simulink model "AlphaBotGyro"  (R2026b)
settings: Solver=FixedStepDiscrete  StopTime=inf  FixedStep=PAR_Sys_AbtastBasis_f64  EnableMultiTasking=on
StopFcn:
  | SpeichereGyroMessung('AlphaBotGyro');
model workspace (MAT data in the model file):
  PAR_AktMot_PWMLKreis_u8 = 60
  PAR_AktMot_PWMRKreis_u8 = 100
  PAR_AktMot_RichtL_u8 = 0
  PAR_AktMot_RichtR_u8 = 0
  PAR_AktMot_Start_f32 = Simulink.Parameter
  PAR_AktMot_Start_f32.Value = 0
  PAR_AktMot_Start_f32.Complexity = 'real'
  PAR_AktMot_Start_f32.Dimensions = [1 1]
  PAR_AktMot_Start_f32.DataType = 'single'
  PAR_RegKrs_TKreis_f64 = 10
  PAR_SenGyr_Abtast_f64 = 0.01
  PAR_SenGyr_NKalib_f64 = 1000
  PAR_Sys_AbtastBasis_f64 = 0.01
  PAR_Sys_Abtast_f64 = 0.01
libraries: arduinolib x6, arduinosensorlib x1
settings Model: SILPILModeSetting=veronly  SimulationMode=external
settings SolverCC: AutoInsertRateTranBlk=on
settings OptimizationCC: DifferentSizesBufferReuse=on  EfficientTunableParamExpr=on  EnhancedBackFolding=on  MaxStackSize=64  OptimizationCustomize=off  OptimizeBlockOrder=speed  PassReuseOutputArgsAs=Individual arguments  RemoveInternalMemoryZeroInit=on  RemoveRootLevelIOMemoryZeroInit=on
settings DebuggingCC: ParameterTunabilityLossMsg=error
settings HardwareCC: ProdHWDeviceType=ARM Compatible->ARM Cortex  ProdLargestAtomicFloat=Double  ProdLargestAtomicInteger=Long
settings SFSimCC: MATLABDynamicMemAlloc=off
settings RTWCC: BuildConfiguration=Faster Runs  Description=Embedded Coder  HardwareBoard=Arduino Uno R4 WiFi  SystemTargetFile=ert.tlc  TLCOptions=-aInlineSetEventsForThisBaseRateFcn=TLC_FALSE -aSuppressMultiTaskScheduler=TLC_FALSE -aRateBasedStepFcn=1  TemplateMakefile=ert_default_tmf  Toolchain=Arduino ARM M4
settings CodeAppCC: ForceParamTrailComments=on  IgnoreCustomStorageClasses=off  InsertBlockDesc=on  OperatorAnnotations=on  SFDataObjDesc=on  SimulinkDataObjDesc=on
settings ERTTargetCC: CombineSignalStateStructs=on  ExtModeAutomaticAllocSize=off  ExtModeIntrfLevel=Level2 - Open  ExtModeMexFile=ext_xcp  ExtModeStaticAlloc=on  SupportContinuousTime=on  SupportVariableSizeSignals=on

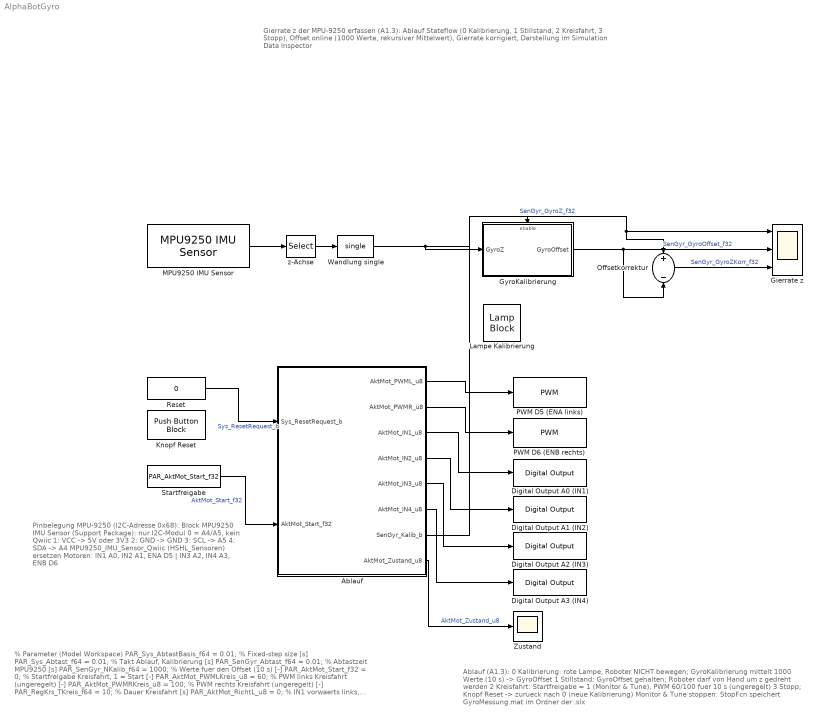
== system AlphaBotGyro ==
  note: % Parameter (Model Workspace)
      | PAR_Sys_AbtastBasis_f64 = 0.01; % Fixed-step size [s]
      | PAR_Sys_Abtast_f64 = 0.01; % Takt Ablauf, Kalibrierung [s]
      | PAR_SenGyr_Abtast_f64 = 0.01; % Abtastzeit MPU9250 [s]
      | PAR_SenGyr_NKalib_f64 = 1000; % Werte fuer den Offset (10 s) [-]
      | PAR_AktMot_Start_f32 = 0; % Startfreigabe Kreisfahrt, 1 = Start [-]
      | PAR_AktMot_PWMLKreis_u8 = 60; % PWM links Kreisfahrt (ungeregelt) [-]
      | PAR_AktMot_PWMRKreis_u8 = 100; % PWM rechts Kreisfahrt (ungeregelt) [-]
      | PAR_RegKrs_TKreis_f64 = 10; % Dauer Kreisfahrt [s]
      | PAR_AktMot_RichtL_u8 = 0; % IN1 vorwaerts links, IN2 = 1 - IN1 [-]
      | PAR_AktMot_RichtR_u8 = 1; % IN3 vorwaerts rechts, IN4 = 1 - IN3 [-]
  note: Gierrate z der MPU-9250 erfassen (A1.3): Ablauf Stateflow (0 Kalibrierung, 1 Stillstand, 2 Kreisfahrt, 3 Stopp), Offset online (1000 Werte, rekursiver Mittelwert), Gierrate korrigiert, Darstellung im Simulation Data Inspector
  note: Pinbelegung MPU-9250 (I2C-Adresse 0x68):
      | Block MPU9250 IMU Sensor (Support Package): nur I2C-Modul 0 = A4/A5, kein Qwiic
      | 1: VCC -> 5V oder 3V3
      | 2: GND -> GND
      | 3: SCL -> A5
      | 4: SDA -> A4
      | MPU9250_IMU_Sensor_Qwiic (HSHL_Sensoren) ersetzen
      | Motoren: IN1 A0, IN2 A1, ENA D5 | IN3 A2, IN4 A3, ENB D6
  note: Ablauf (A1.3):
      | 0 Kalibrierung: rote Lampe, Roboter NICHT bewegen; GyroKalibrierung mittelt 1000 Werte (10 s) -> GyroOffset
      | 1 Stillstand: GyroOffset gehalten; Roboter darf von Hand um z gedreht werden
      | 2 Kreisfahrt: Startfreigabe = 1 (Monitor & Tune), PWM 60/100 fuer 10 s (ungeregelt)
      | 3 Stopp; Knopf Reset -> zurueck nach 0 (neue Kalibrierung)
      | Monitor & Tune stoppen: StopFcn speichert GyroMessung.mat im Ordner der .slx
  Ablauf : Stateflow chart  TreatAsAtomicUnit=on
  Digital Output A0 (IN1) : arduinolib/Digital Output  pinNumber=14  Direction=output  blockPlatform=arduino
  Digital Output A1 (IN2) : arduinolib/Digital Output  pinNumber=15  Direction=output  blockPlatform=arduino
  Digital Output A2 (IN3) : arduinolib/Digital Output  pinNumber=16  Direction=output  blockPlatform=arduino
  Digital Output A3 (IN4) : arduinolib/Digital Output  pinNumber=17  Direction=output  blockPlatform=arduino
  Gierrate z : Scope  NumInputPorts=3
  GyroKalibrierung : Subsystem  TreatAsAtomicUnit=on
  Knopf Reset : PushButtonBlock  ButtonText=Reset  IconOnColor=[0.0, 0.39215686274509803, 0.0]  IconOffColor=[0.0, 1.0, 0.0]
  Lampe Kalibrierung : LampBlock  LabelPosition=Hide  DefaultColor=[192.0, 192.0, 192.0]
  MPU9250 IMU Sensor : arduinosensorlib/MPU9250 IMU Sensor  I2CModule=0  SlaveAddress=0x68  Accel=off  AngularRate=on  Ak8963Field=off  Temperature=off  Status=off  EulerAngles=off  Quat=off  Timestamp=off  AccelRange=2G  Acceldlpf=218.1 Hz  GyroRange=250 dps  Gyrodlpf=41 Hz  DmpOdr=200 Hz  spf=1  SampleTime=PAR_SenGyr_Abtast_f64  QueueSizeFactor=1
  Offsetkorrektur : Sum  Inputs=+-
  PWM D5 (ENA links) : arduinolib/PWM  pinNumber=5  frequencyType=Default  desiredFrequency=490.2  achievableFrequency=490.2
  PWM D6 (ENB rechts) : arduinolib/PWM  pinNumber=6  frequencyType=Default  desiredFrequency=490.2  achievableFrequency=490.2
  Reset : Constant  Value=0  OutDataTypeStr=boolean  SampleTime=PAR_Sys_Abtast_f64
  Startfreigabe : Constant  Value=PAR_AktMot_Start_f32  OutDataTypeStr=single  SampleTime=PAR_Sys_Abtast_f64
  Wandlung single : DataTypeConversion  OutDataTypeStr=single  SaturateOnIntegerOverflow=off  RndMeth=Floor
  Zustand : Scope
  z-Achse : Selector  NumberOfDimensions=2  InputPortWidth=3  IndexOptions=Index vector (dialog),Index vector (dialog)  Indices=3,1  OutputSizes=1
  wires:
  MPU9250 IMU Sensor/1 -> z-Achse/1
  z-Achse/1 -> Wandlung single/1
  Wandlung single/1 -> Offsetkorrektur/1, Gierrate z/1, GyroKalibrierung/1(GyroZ)  "SenGyr_GyroZ_f32"
  GyroKalibrierung/1(GyroOffset) -> Offsetkorrektur/2, Gierrate z/2  "SenGyr_GyroOffset_f32"
  Offsetkorrektur/1 -> Gierrate z/3  "SenGyr_GyroZKorr_f32"
  Reset/1 -> Ablauf/1(Sys_ResetRequest_b)  "Sys_ResetRequest_b"
  Startfreigabe/1 -> Ablauf/2(AktMot_Start_f32)  "AktMot_Start_f32"
  Ablauf/1(AktMot_PWML_u8) -> PWM D5 (ENA links)/1
  Ablauf/2(AktMot_PWMR_u8) -> PWM D6 (ENB rechts)/1
  Ablauf/3(AktMot_IN1_u8) -> Digital Output A0 (IN1)/1
  Ablauf/4(AktMot_IN2_u8) -> Digital Output A1 (IN2)/1
  Ablauf/5(AktMot_IN3_u8) -> Digital Output A2 (IN3)/1
  Ablauf/6(AktMot_IN4_u8) -> Digital Output A3 (IN4)/1
  Ablauf/7(SenGyr_Kalib_b) -> GyroKalibrierung/Enable
  Ablauf/8(AktMot_Zustand_u8) -> Zustand/1  "AktMot_Zustand_u8"

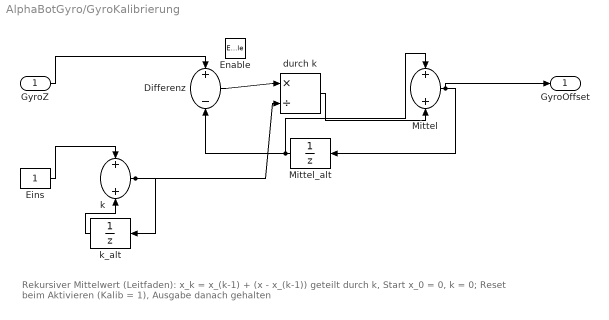
== system AlphaBotGyro/GyroKalibrierung ==
  note: Rekursiver Mittelwert (Leitfaden): x_k = x_(k-1) + (x - x_(k-1)) geteilt durch k, Start x_0 = 0, k = 0; Reset beim Aktivieren (Kalib = 1), Ausgabe danach gehalten
  GyroZ : Inport
  Enable : EnablePort  StatesWhenEnabling=reset
  Differenz : Sum  Inputs=+-
  Eins : Constant  OutDataTypeStr=single
  Mittel : Sum
  Mittel_alt : UnitDelay  SampleTime=-1
  durch k : Product  Inputs=*/
  k : Sum
  k_alt : UnitDelay  SampleTime=-1
  GyroOffset : Outport  InitialOutput=0
  wires:
  GyroZ/1 -> Differenz/1
  Mittel_alt/1 -> Differenz/2, Mittel/1
  Differenz/1 -> durch k/1
  Eins/1 -> k/1
  k_alt/1 -> k/2
  k/1 -> k_alt/1, durch k/2
  durch k/1 -> Mittel/2
  Mittel/1 -> Mittel_alt/1, GyroOffset/1

== stateflow chart AlphaBotGyro/Ablauf ==
  settings: updateMethod=DISCRETE  sampleTime=PAR_Sys_Abtast_f64
  state Kalibrierung
    entry:
    AktMot_PWML_u8 = uint8(0);
    AktMot_PWMR_u8 = uint8(0);
    AktMot_IN1_u8 = uint8(0);
    AktMot_IN2_u8 = uint8(0);
    AktMot_IN3_u8 = uint8(0);
    AktMot_IN4_u8 = uint8(0);
    SenGyr_Kalib_b = true;
    AktMot_Zustand_u8 = uint8(0);
    during:
    SenGyr_Kalib_b = ~Sys_ResetRequest_b;
    Kalibrierung -> Kalibrierung [order 1] : [Sys_ResetRequest_b]
  state Stillstand
    entry:
    AktMot_PWML_u8 = uint8(0);
    AktMot_PWMR_u8 = uint8(0);
    AktMot_IN1_u8 = uint8(0);
    AktMot_IN2_u8 = uint8(0);
    AktMot_IN3_u8 = uint8(0);
    AktMot_IN4_u8 = uint8(0);
    SenGyr_Kalib_b = false;
    AktMot_Zustand_u8 = uint8(1);
  state Kreisfahrt
    entry:
    AktMot_PWML_u8 = PAR_AktMot_PWMLKreis_u8;
    AktMot_PWMR_u8 = PAR_AktMot_PWMRKreis_u8;
    AktMot_IN1_u8 = PAR_AktMot_RichtL_u8;
    AktMot_IN2_u8 = uint8(1) - PAR_AktMot_RichtL_u8;
    AktMot_IN3_u8 = PAR_AktMot_RichtR_u8;
    AktMot_IN4_u8 = uint8(1) - PAR_AktMot_RichtR_u8;
    SenGyr_Kalib_b = false;
    AktMot_Zustand_u8 = uint8(2);
  state Stopp
    entry:
    AktMot_PWML_u8 = uint8(0);
    AktMot_PWMR_u8 = uint8(0);
    AktMot_IN1_u8 = uint8(0);
    AktMot_IN2_u8 = uint8(0);
    AktMot_IN3_u8 = uint8(0);
    AktMot_IN4_u8 = uint8(0);
    SenGyr_Kalib_b = false;
    AktMot_Zustand_u8 = uint8(3);
  (default) -> Kalibrierung
  Stillstand -> Kalibrierung [order 1] : [Sys_ResetRequest_b]
  Kalibrierung -> Stillstand [order 1] : [after(PAR_SenGyr_NKalib_f64,tick)]
  Kreisfahrt -> Kalibrierung [order 1] : [Sys_ResetRequest_b]
  Stillstand -> Kreisfahrt [order 2] : [AktMot_Start_f32 >= 1]
  Stopp -> Kalibrierung : [Sys_ResetRequest_b]
  Kreisfahrt -> Stopp [order 2] : [after(PAR_RegKrs_TKreis_f64,sec)]
  data: Sys_ResetRequest_b input boolean; AktMot_Start_f32 input single; AktMot_PWML_u8 output uint8; AktMot_PWMR_u8 output uint8; AktMot_IN1_u8 output uint8; AktMot_IN2_u8 output uint8; AktMot_IN3_u8 output uint8; AktMot_IN4_u8 output uint8; SenGyr_Kalib_b output boolean; AktMot_Zustand_u8 output uint8; PAR_SenGyr_NKalib_f64 parameter; PAR_RegKrs_TKreis_f64 parameter; PAR_AktMot_PWMLKreis_u8 parameter; PAR_AktMot_PWMRKreis_u8 parameter; PAR_AktMot_RichtL_u8 parameter; PAR_AktMot_RichtR_u8 parameter
